simulink model "untitled"  (R2023b)
settings: Solver=VariableStepAuto  StartTime=0.0  StopTime=0.1  RelTol=1e-3
libraries: spsVoltageMeasurementLib x9, spsThyristorLib x6, spsACVoltageSourceLib x5, spsCurrentMeasurementLib x2, spsSeriesRLCBranchLib x2, spsDCVoltageSourceLib x1, spsGroundLib x1, sps_lib x1
settings Model: Creator=hafeizhou  LastModifiedBy=hafeizhou

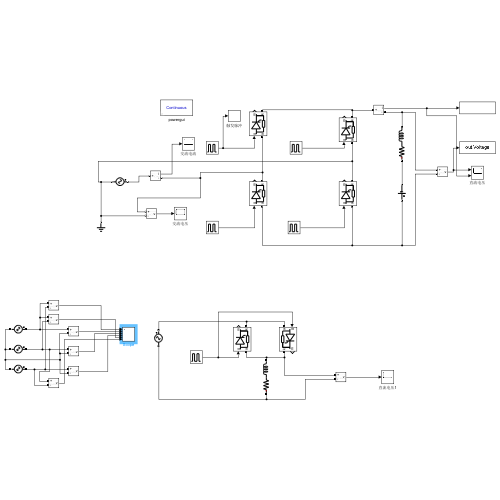
[thumbnail: Simulink's stored preview of the top-level diagram]
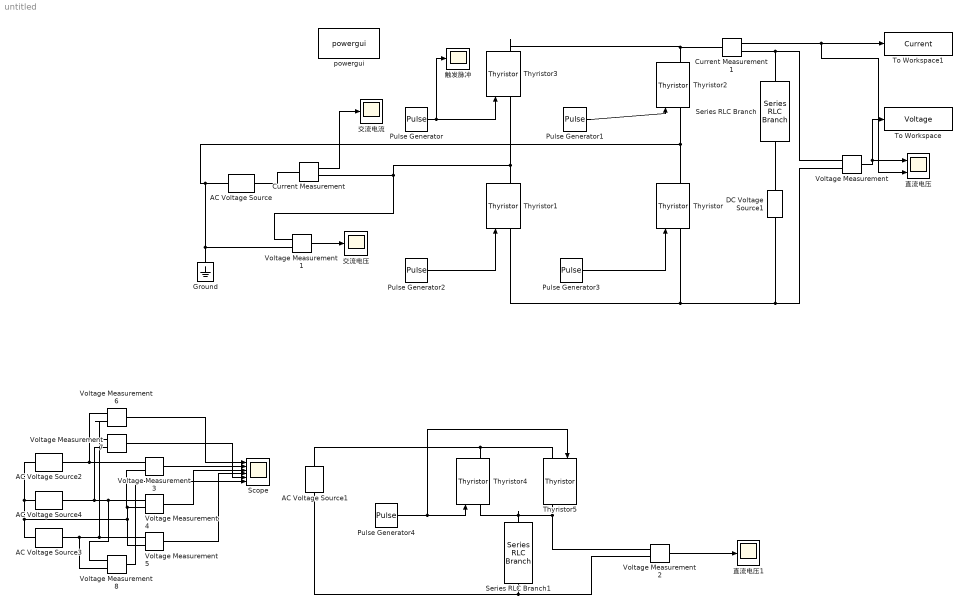
== system untitled ==
  AC Voltage Source : spsACVoltageSourceLib/AC Voltage Source  Amplitude=20  Phase=0  Frequency=50  SampleTime=0  Measurements=None  BusType=swing  Pref=10e3  Qref=0  Qmin=-inf  Qmax=+inf
  AC Voltage Source1 : spsACVoltageSourceLib/AC Voltage Source  Amplitude=20  Phase=0  Frequency=50  SampleTime=0  Measurements=None  BusType=swing  Pref=10e3  Qref=0  Qmin=-inf  Qmax=+inf
  AC Voltage Source2 : spsACVoltageSourceLib/AC Voltage Source  Amplitude=20  Phase=0  Frequency=50  SampleTime=0  Measurements=None  BusType=swing  Pref=10e3  Qref=0  Qmin=-inf  Qmax=+inf
  AC Voltage Source3 : spsACVoltageSourceLib/AC Voltage Source  Amplitude=20  Phase=120  Frequency=50  SampleTime=0  Measurements=None  BusType=swing  Pref=10e3  Qref=0  Qmin=-inf  Qmax=+inf
  AC Voltage Source4 : spsACVoltageSourceLib/AC Voltage Source  Amplitude=20  Phase=240  Frequency=50  SampleTime=0  Measurements=None  BusType=swing  Pref=10e3  Qref=0  Qmin=-inf  Qmax=+inf
  Current Measurement : spsCurrentMeasurementLib/Current Measurement  PhasorSimulation=off  OutputType=Complex  PSBequivalent=0
  Current Measurement1 : spsCurrentMeasurementLib/Current Measurement  PhasorSimulation=off  OutputType=Complex  PSBequivalent=0
  DC Voltage Source1 : spsDCVoltageSourceLib/DC Voltage Source  Amplitude=20  Measurements=Voltage
  Ground : spsGroundLib/Ground  LConnTagsString=a
  Pulse Generator : DiscretePulseGenerator  PulseType=Time based  Period=0.02  PulseWidth=20  PhaseDelay=0.009167
  Pulse Generator1 : DiscretePulseGenerator  PulseType=Time based  Period=0.02  PulseWidth=20  PhaseDelay=0.019167
  Pulse Generator2 : DiscretePulseGenerator  PulseType=Time based  Period=0.02  PulseWidth=20  PhaseDelay=0.019167
  Pulse Generator3 : DiscretePulseGenerator  PulseType=Time based  Period=0.02  PulseWidth=20  PhaseDelay=0.009167
  Pulse Generator4 : DiscretePulseGenerator  PulseType=Time based  Period=0.01  PulseWidth=10  PhaseDelay=0.005
  Scope : Scope  NumInputPorts=6
  Series RLC Branch : spsSeriesRLCBranchLib/Series RLC Branch  LConnTagsString=__new0  RConnTagsString=__new0  BranchType=RL  Resistance=8.5  Inductance=0.004  SetiL0=off  InitialCurrent=0  Capacitance=1e-6  Setx0=off  InitialVoltage=0  Measurements=None
  Series RLC Branch1 : spsSeriesRLCBranchLib/Series RLC Branch  LConnTagsString=__new0  RConnTagsString=__new0  BranchType=RL  Resistance=8.5  Inductance=0.004  SetiL0=off  InitialCurrent=0  Capacitance=1e-6  Setx0=off  InitialVoltage=0  Measurements=None
  Thyristor{,1..5} (6 alike) : spsThyristorLib/Thyristor  Ron=0.001  Lon=0  Vf=0.8  IC=0  Rs=500  Cs=250e-9  Measurements=on
  To Workspace : ToWorkspace  VariableName=Voltage  SaveFormat=Timeseries  SampleTime=-1
  To Workspace1 : ToWorkspace  VariableName=Current  SaveFormat=Timeseries  SampleTime=-1
  Voltage Measurement{,1..8} (9 alike) : spsVoltageMeasurementLib/Voltage Measurement  PhasorSimulation=off  OutputType=Complex  PSBequivalent=0
  powergui : sps_lib/powergui  Priority=1  SimulationMode=Continuous  SampleTime=50e-6  frequency=60  Iterations=50  frequencyindice=50  Pbase=100e6  ErrMax=1e-4  UnitsV=kV  UnitsW=MW  buscounter=0  FunctionMessages=off  echomessages=off  EnableUseOfTLC=off  CurrentSourceSwitches=off  DisableSnubberDevices=off  DisableRonSwitches=off  DisableVfSwitches=off  DisplayEquations=off  AutomaticDiscreteSolvers=off  SolverType=Tustin/Backward Euler (TBE)  Interpol=off  ExternalGateDelay=off  methode=off  Ts=100  x0status=blocks  SPID=on  SwTol=0  HookPort=off  NonlinearTolerance=1e-4  nMaxIteration=100  ContinueOnMaxIteration=off  RestoreLinks=warning  ResistiveCurrentMeasurement=off  Frange=[0:2:500]  Ylog=off  Xlog=on  ShowGrid=off  save=off  variable=ZData  structure=0  ZoomFFT=off  StartTime=0.0  cycles=1  DisplayStyle=1  fundamental=60  FreqAxis=off  MaxFrequency=1000  frequencyindicesteady=1  RmsSteady=1  display=off
  交流电压 : Scope
  交流电流 : Scope
  直流电压 : Scope  NumInputPorts=2
  直流电压1 : Scope
  触发脉冲 : Scope
  wires:
  Pulse Generator/1 -> 触发脉冲/1, Thyristor3/1
  Pulse Generator3/1 -> Thyristor/1
  Voltage Measurement/1 -> To Workspace/1, 直流电压/1
  Pulse Generator1/1 -> Thyristor2/1
  Pulse Generator2/1 -> Thyristor1/1
  Voltage Measurement1/1 -> 交流电压/1
  Current Measurement/1 -> 交流电流/1
  Current Measurement1/1 -> 直流电压/2, To Workspace1/1
  Voltage Measurement2/1 -> 直流电压1/1
  Pulse Generator4/1 -> Thyristor5/1, Thyristor4/1
  Voltage Measurement3/1 -> Scope/2
  Voltage Measurement4/1 -> Scope/3
  Voltage Measurement6/1 -> Scope/1
  Voltage Measurement5/1 -> Scope/4
  Voltage Measurement7/1 -> Scope/5
  Voltage Measurement8/1 -> Scope/6
  connections:
  Thyristor/RConn1 -- Thyristor2/LConn1 -- Voltage Measurement1/LConn2 -- Ground/LConn1 -- AC Voltage Source/LConn1
  Thyristor/LConn1 -- DC Voltage Source1/RConn1 -- Voltage Measurement/LConn2 -- Thyristor1/LConn1
  Voltage Measurement1/LConn1 -- Current Measurement/RConn1 -- Thyristor3/LConn1 -- Thyristor1/RConn1
  Thyristor3/RConn1 -- Current Measurement1/LConn1 -- Thyristor2/RConn1
  Current Measurement/LConn1 -- AC Voltage Source/RConn1
  Current Measurement1/RConn1 -- Series RLC Branch/RConn1 -- Voltage Measurement/LConn1
  Series RLC Branch/LConn1 -- DC Voltage Source1/LConn1
  Thyristor4/RConn1 -- AC Voltage Source1/RConn1 -- Thyristor5/LConn1
  Thyristor5/RConn1 -- Voltage Measurement2/LConn1 -- Thyristor4/LConn1 -- Series RLC Branch1/RConn1
  AC Voltage Source1/LConn1 -- Voltage Measurement2/LConn2 -- Series RLC Branch1/LConn1
  AC Voltage Source3/RConn1 -- Voltage Measurement8/LConn2 -- Voltage Measurement6/LConn2 -- Voltage Measurement5/LConn1
  Voltage Measurement4/LConn1 -- Voltage Measurement8/LConn1 -- Voltage Measurement7/LConn2 -- AC Voltage Source4/RConn1
  AC Voltage Source2/RConn1 -- Voltage Measurement7/LConn1 -- Voltage Measurement6/LConn1 -- Voltage Measurement3/LConn1
  AC Voltage Source2/LConn1 -- AC Voltage Source3/LConn1 -- Voltage Measurement4/LConn2 -- Voltage Measurement3/LConn2 -- Voltage Measurement5/LConn2 -- AC Voltage Source4/LConn1
